simulink model "BMS_Estimator_Test"  (R2025b)
settings: Solver=FixedStepDiscrete  StartTime=0.0  StopTime=1  FixedStep=Ts  RelTol=1e-3
InitFcn:
  | init_BMS
undefined symbols (not defined in the file): Ts
libraries: BMS_Library x1
settings Model: Creator=Khadija  LastModifiedBy=Khadija

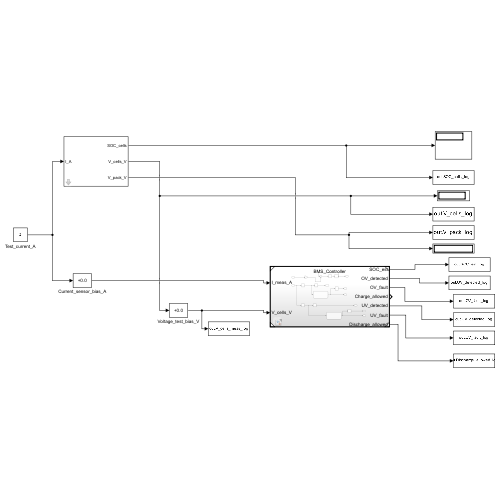
[thumbnail: Simulink's stored preview of the top-level diagram]
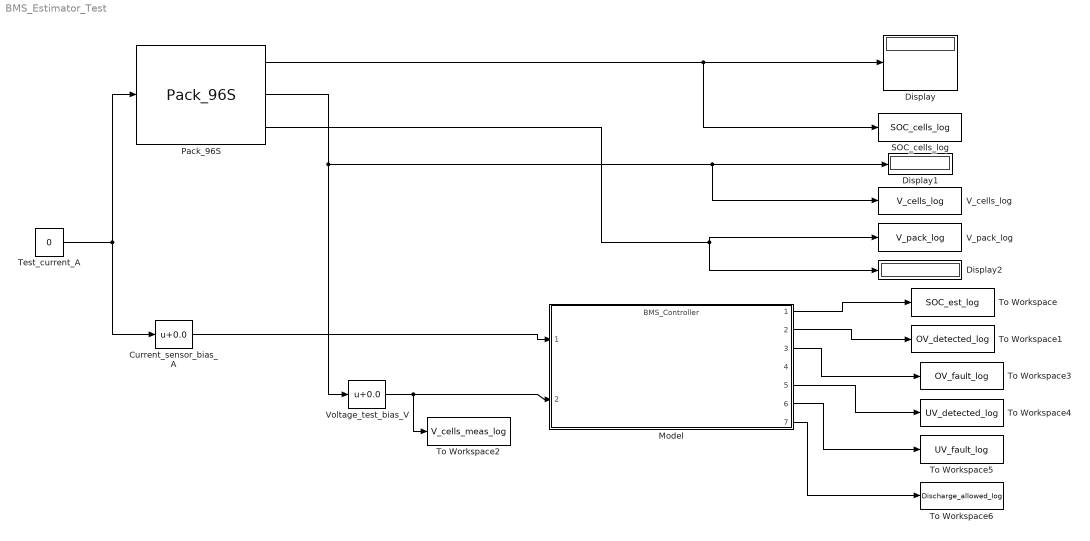
== system BMS_Estimator_Test ==
  Current_sensor_bias_A : Bias  Bias=0.0  SaturateOnIntegerOverflow=off
  Display : Display
  Display1 : Display
  Display2 : Display
  Model : ModelReference  ModelNameDialog=BMS_Controller  SimulationMode=Normal  ModelReferenceVersion=1.26
  Pack_96S : BMS_Library/Pack_96S  SOC_init_pack=SOC0_pack
  SOC_cells_log : ToWorkspace  VariableName=SOC_cells_log  SaveFormat=Timeseries  SampleTime=-1
  Test_current_A : Constant  Value=0  SampleTime=Ts
  To Workspace : ToWorkspace  VariableName=SOC_est_log  SaveFormat=Timeseries  SampleTime=-1
  To Workspace1 : ToWorkspace  VariableName=OV_detected_log  SaveFormat=Timeseries  SampleTime=-1
  To Workspace2 : ToWorkspace  VariableName=V_cells_meas_log  SaveFormat=Timeseries  SampleTime=-1
  To Workspace3 : ToWorkspace  VariableName=OV_fault_log  SaveFormat=Timeseries  SampleTime=-1
  To Workspace4 : ToWorkspace  VariableName=UV_detected_log  SaveFormat=Timeseries  SampleTime=-1
  To Workspace5 : ToWorkspace  VariableName=UV_fault_log  SaveFormat=Timeseries  SampleTime=-1
  To Workspace6 : ToWorkspace  VariableName=Discharge_allowed_log  SaveFormat=Timeseries  SampleTime=-1
  V_cells_log : ToWorkspace  VariableName=V_cells_log  SaveFormat=Timeseries  SampleTime=-1
  V_pack_log : ToWorkspace  VariableName=V_pack_log  SaveFormat=Timeseries  SampleTime=-1
  Voltage_test_bias_V : Bias  Bias=0.0  SaturateOnIntegerOverflow=off
  wires:
  Test_current_A/1 -> Current_sensor_bias_A/1, Pack_96S/1
  Pack_96S/1 -> SOC_cells_log/1, Display/1
  Pack_96S/2 -> Voltage_test_bias_V/1, Display1/1, V_cells_log/1
  Pack_96S/3 -> Display2/1, V_pack_log/1
  Model/1 -> To Workspace/1
  Current_sensor_bias_A/1 -> Model/1
  Model/2 -> To Workspace1/1
  Voltage_test_bias_V/1 -> Model/2, To Workspace2/1
  Model/3 -> To Workspace3/1
  Model/5 -> To Workspace4/1
  Model/6 -> To Workspace5/1
  Model/7 -> To Workspace6/1
